simulink model "S_Tek_NDI_6DOF"  (R2025b)
settings: Solver=ode4  StartTime=0.0  StopTime=5  FixedStep=0.001  RelTol=1e-3
undefined symbols (not defined in the file): X, Y, Z
libraries: sm_lib x15, nesl_utility x13, instrumentseriallib x3, svdutilitieslib x2, sharedtransform x1, aerolibanimutils x1
(part 2 of 2)

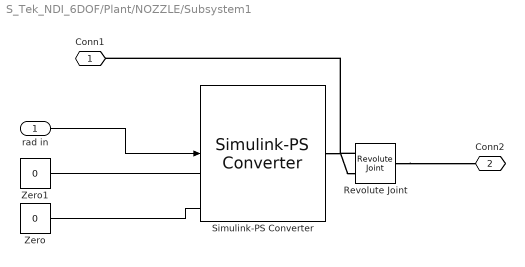
== system S_Tek_NDI_6DOF/Plant/NOZZLE/Subsystem1 ==
  rad in : Inport
  Revolute Joint : sm_lib/Joints/Revolute Joint  JointMode=Normal  CompositeWrenchDir=FollowerOnBase  CompositeWrenchFrame=BaseFrame  SenseConstraintForce=off  SenseConstraintTorque=off  SenseTotalForce=off  SenseTotalTorque=off  PositionTargetSpecify=off  PositionTargetPriority=High  PositionTargetValue=0  PositionTargetValueUnits=deg  VelocityTargetSpecify=off  VelocityTargetPriority=High  VelocityTargetValue=0  VelocityTargetValueUnits=deg/s  EquilibriumPosition=0  EquilibriumPositionUnits=deg  SpringStiffness=0  SpringStiffnessUnits=N*m/deg  DampingCoefficient=0  DampingCoefficientUnits=N*m/(deg/s)  LowerLimitSpecify=off  LowerLimitBound=-90  LowerLimitBoundUnits=deg  LowerLimitStiffness=1e4  LowerLimitStiffnessUnits=N*m/deg  LowerLimitDamping=10  LowerLimitDampingUnits=N*m/(deg/s)  LowerLimitTransitionRegionWidth=0.1  LowerLimitTransitionRegionWidthUnits=deg  UpperLimitSpecify=off  UpperLimitBound=90  UpperLimitBoundUnits=deg  UpperLimitStiffness=1e4  UpperLimitStiffnessUnits=N*m/deg  UpperLimitDamping=10  UpperLimitDampingUnits=N*m/(deg/s)  UpperLimitTransitionRegionWidth=0.1  UpperLimitTransitionRegionWidthUnits=deg  TorqueActuationMode=ComputedTorque  MotionActuationMode=InputMotion  SensePosition=off  SenseVelocity=off  SenseAcceleration=off  SenseTorqueForce=off  SenseLowerLimitTorqueForce=off  SenseUpperLimitTorqueForce=off
  Simulink-PS Converter : nesl_utility/Simulink-PS Converter  PhysicalDomain=network_engine_domain  SubClassName=ps_input  LeftPortType=input  RightPortType=output  PseudoPeriodic=off  Frequencies=[]  NoiseDistribution=none  NoiseParameters=[]  Unit=1  AffineConversion=off  FilteringAndDerivatives=filter  SimscapeFilterOrder=2  InputFilterTimeConstant=0.001  UdotUserProvided=2
  Zero : Constant  Value=0  OutDataTypeStr=Inherit: Inherit via back propagation
  Zero1 : Constant  Value=0  OutDataTypeStr=Inherit: Inherit via back propagation
  Conn1 : PMIOPort  Side=Left
  Conn2 : PMIOPort  Port=2  Side=Right
  wires:
  Zero/1 -> ?
  Zero1/1 -> ?
  rad in/1 -> Simulink-PS Converter/1
  connections:
  Simulink-PS Converter/RConn1 -- Revolute Joint/LConn2
  Revolute Joint/LConn1 -- Conn1/RConn1
  Revolute Joint/RConn1 -- Conn2/RConn1

== matlab function S_Tek_NDI_6DOF/Guiadance/MATLAB Function1 ==
  settings: updateMethod=DISCRETE
  data: z input; v_ref output; t input; motor_status output
function [v_ref, motor_status] = landing_logic(z, t)
%#codegen

% 1. ÇIKIŞLARA VARSAYILAN DEĞERLER
v_ref = 0.0;
motor_status = 1.0;

% Kalıcı değişkenler
persistent stage;
persistent t_reach_5m;

if isempty(stage)
    stage = 1;         % Başlangıç: Tırmanış fazı
    t_reach_5m = 0.0;
end

% Parametreler
z_target_hover  = 5.0; % [m] Hedef hover irtifası
t_hold_duration = 5.0; % [sn] Havada askıda kalma süresi (5 saniye)
v_climb         = 2; % [m/s] Tırmanış hızı

switch stage
    case 1
        % --- AŞAMA 1: 2 METREDEN 5 METREYE TIRMANIŞ ---
        v_ref = v_climb;
        motor_status = 1.0;
        
        if z >= (z_target_hover - 0.05) % 4.95 metreye ulaşıldığında
            stage = 2;
            t_reach_5m = t; % 5 metreye ulaşılan anın zamanını kaydet
        end
        
    case 2
        % --- AŞAMA 2: 5 METREDE 5 SANİYE HOVER ---
        v_ref = 0.0;        % 0 m/s hız referansı
        motor_status = 1.0; % Motorlar aktif
        
        if (t - t_reach_5m) >= t_hold_duration % 5 saniye tamamlandı mı?
            stage = 3;      % Görev bitti, kapatmaya geç
        end
        
    case 3
        % --- AŞAMA 3: GÖREV TAMAMLANDI (SİSTEM KAPALI) ---
        v_ref = 0.0;
        motor_status = 0.0; % Valfleri ve itkiyi tamamen kapat
        
    otherwise
        v_ref = 0.0;
        motor_status = 0.0;
end

== matlab function S_Tek_NDI_6DOF/Guiadance/MATLAB Function ==
  settings: updateMethod=DISCRETE
  data: z input; vz input; v_ref output; z_activation input; z_cutoff input; motor_status output; mission_mode input
function [v_ref, motor_status] = landing_logic(z, vz, z_activation, z_cutoff, mission_mode)
%#codegen
% z             : İrtifa [m], + yukarı
% vz            : Düşey hız [m/s], + yukarı, - aşağı (Düşerken negatiftir)
% z_activation  : Aktivasyon irtifası (Burası artık kesinlikle 5.0)
% z_cutoff      : İtki kesme irtifası [m] (Örn: 0.08)
% mission_mode  : 1 = Landing Modu, 2 = Hover Modu, Diğer = Motor Kapalı

% Kalıcı (Persistent) Değişken: Sistem ilk açıldığında serbest düşüş hızını kilitlemek için
persistent v_entry_speed;
if isempty(v_entry_speed)
    v_entry_speed = -8.86; % Teorik başlangıç tahmini (9 metreden düşen 33 kg için)
end

% Negatif irtifa koruması
if z < 0.0
    z = 0.0;
end

% =========================================================
% YENİ AGRESİF PARAMETRELER (5 METRE SERBEST DÜŞÜŞ SENARYOSU)
% =========================================================
z_flare_start = 4.90;       % [m] Sistem açılır açılmaz (5m) frenleme başlasın diye pay
z_touch_zone  = 0.25;       % [m] Son dokunuş bölgesi yüksekliği
v_land_touch  = -0.15;      % [m/s] Hedeflenen güvenli temas hızı (Max 0.20'nin altında)
vz_cutoff_min = -0.25;      % [m/s] Motor kesme için maksimum dikey hız
vz_cutoff_max =  0.05;      % [m/s] Motor kesme için minimum dikey hız

% =========================================================
% HOVER BÖLGESİ PARAMETRELERİ (MISSION_MODE == 2)
% =========================================================
z_hover_target = 5.0;       % [m] Hedeflenen hover yüksekliği
z_hover_start  = 2.0;       % [m] Hover modunun başladığı zemin yüksekliği
v_climb        = 0.50;      % [m/s] Güvenli tırmanış hızı referansı (Pozitif)

% =========================================================
% ANA MANTIĞIN ÇALIŞTIRILMASI
% =========================================================
if mission_mode == 1
    % LANDING MODU
    if z > z_activation
        % 5 metrenin üstündeyiz: Tam serbest düşüş, motorlar kapalı
        v_ref = 0.0;
        motor_status = 0.0;
        v_entry_speed = vz; % Sistem devreye girene kadar anlık hızı hafızada tut
        
    elseif (z <= z_cutoff) && (vz >= vz_cutoff_min) && (vz <= vz_cutoff_max)
        % Yere ulaşıldı ve hız güvenli sınırda: Motorları tamamen kapat
        v_ref = 0.0;
        motor_status = 0.0;
        
    else
        % AKTİF ACİL FRENLEME BÖLGESİ (z <= 5m)
        motor_status = 1.0; % Motorlar hemen aktif!
        
        if z > z_flare_start
            % Tetiklenmenin ilk saliseleri için referansı giriş hızına eşitle
            v_cmd = v_entry_speed;
            
        elseif z > z_touch_zone
            % Dinamik Rampalama:
            % Araç 5 metreden girdikten sonra hızı v_entry_speed'den v_land_touch'a lineer düşürür
            denom = z_flare_start - z_touch_zone;
            if denom < 1e-4, denom = 1e-4; end
            
            ratio = (z - z_touch_zone) / denom;
            ratio = max(min(ratio, 1.0), 0.0); % 0 ile 1 arasına sıkıştır
            
            % Frenleme referans hızı hesabı
            v_cmd = v_land_touch + ratio * (v_entry_speed - v_land_touch);
        else
            % Son 25 cm: Hedeflenen 0.15 m/s hızla yumuşak dokunuş yap
            v_cmd = v_land_touch;
        end
        
        v_ref = v_cmd;
    end
    
elseif mission_mode == 2
    % =========================================================
    % HOVER MODU EKLENTİSİ
    % =========================================================
    motor_status = 1.0; % Motorlar hover için kesinlikle aktif olmalı
    
    if z >= z_hover_target
        % Araç 5 metreye ulaştı veya üstünde: Düşey hız referansını 0 yap (Sabit kal)
        v_ref = 0.0;
    elseif z <= z_hover_start
        % Araç henüz 2 metrenin altında veya sınırda: Maksimum tırmanış hızı ver
        v_ref = v_climb;
    else
        % 2 metre ile 5 metre arasında dinamik yaklaşım (Yumuşak duruş için)
        % Hedefe yaklaştıkça hız referansını lineer olarak azaltarak sönümleme yapıyoruz
        denom_hover = z_hover_target - z_hover_start;
        if denom_hover < 1e-4, denom_hover = 1e-4; end
        
        % Hedefe olan mesafe oranı (5 metreye yaklaştıkça ratio_hover -> 0 olur)
        ratio_hover = (z_hover_target - z) / denom_hover;
        ratio_hover = max(min(ratio_hover, 1.0), 0.0);
        
        % Hız referansı (Hedefe yaklaştıkça 0'a yaklaşır, 2 metreye yaklaştıkça v_climb olur)
        v_ref = ratio_hover * v_climb;
    end
    
    % Hover modundayken de v_entry_speed'i güncel tutuyoruz ki landing moduna ani 
    % bir geçiş olursa hafıza hatalı kalmasın.
    v_entry_speed = vz;

else
    % Diğer modlar (Motor Off vb.)
    v_ref = 0.0;
    motor_status = 0.0;
    v_entry_speed = vz; % Aktif değilken hızı takip etmeye devam et
end
end

== matlab function S_Tek_NDI_6DOF/Guiadance/MATLAB Function2 ==
  settings: updateMethod=DISCRETE
  data: h input; v_ref_m_sn output; Vz_current input; mode output
function [v_ref_m_sn, mode] = Guidance_Profile(h, Vz_current)
%#codegen

    % 1. Çıkış değişkenlerine en başta varsayılan değerleri tanımlayın
    v_ref_m_sn = 0.0;
    mode       = 0.0;

    % Parametreler
    a_des   = 5.20;
    h_flare = 0.60;
    v_td    = 0.20;
    h_act   = 6.74;
    h_touch = 1;

    persistent flight_state;
    if isempty(flight_state)
        flight_state = 0;
    end

    % Durum geçişleri
    if flight_state == 0
        if (h <= h_act) && (Vz_current < -0.5)
            flight_state = 1;
        end
    elseif flight_state == 1
        if h <= h_touch
            flight_state = 2;
        end
    end

    % Çıktı atamaları
    switch flight_state
        case 0  % Serbest Düşüş
            mode       = 0.0;
            v_ref_m_sn = Vz_current;

        case 1  % Aktif Frenleme & Flare
            mode = 1.0;
            if h > h_flare
                delta_h = h - h_flare;
                if delta_h < 0.0
                    delta_h = 0.0;
                end
                v_ref_m_sn = -sqrt((v_td^2) + 2.0 * a_des * delta_h);
            else
                v_ref_m_sn = -v_td;
            end

        case 2  % Touchdown / Kapanma
            mode       = 0.0;
            v_ref_m_sn = 0.0;

        otherwise % Olası tanımlanmamış durumlar için koruma
            mode       = 0.0;
            v_ref_m_sn = 0.0;
    end
end
